simulink model "model_20ms"  (R2026a)
settings: Solver=VariableStepAuto
undefined symbols (not defined in the file): MIO, National_Instruments, PCI
libraries: sldrtlib x2, simulink x1
settings Model: Creator=acsdc  LastModifiedBy=acsdc

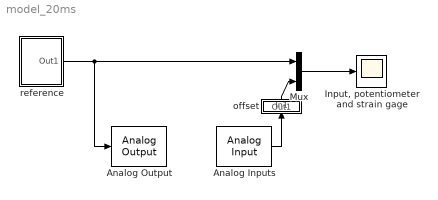
== system model_20ms ==
  Analog Inputs : sldrtlib/Analog Input  SampleTime=0.02  MaxMissedTicks=1000  ShowMissedTicks=off  YieldWhenWaiting=off  DrvName=National_Instruments/PCI-MIO-16E-4  DrvAddress=4294967295  DrvOptions=[0 0 0 0 0 0]  Channels=1:4  RangeMode=1  VoltRange=1  DataType=1
      settings: AttributesFormatString=National Instruments\nPCI-MIO-16E-4 [auto]
  Analog Output : sldrtlib/Analog Output  SampleTime=0.02  MaxMissedTicks=1000  ShowMissedTicks=off  YieldWhenWaiting=off  DrvName=National_Instruments/PCI-MIO-16E-4  DrvAddress=4294967295  DrvOptions=[0 0 0 0 0 0]  Channels=1  RangeMode=1  VoltRange=1  InitialValue=0  FinalValue=0
      settings: AttributesFormatString=National Instruments\nPCI-MIO-16E-4 [auto]
  "Input, potentiometer and strain gage" : Scope
      settings: DataLoggingSaveFormat=Array
  Mux : Mux  Inputs=2
  offset : Subsystem
  reference : Subsystem
  wires:
  Mux/1 -> "Input, potentiometer and strain gage"/1
  offset/1(Out1) -> Mux/2
  reference/1(Out1) -> Analog Output/1, Mux/1
  Analog Inputs/1 -> offset/1(In1)

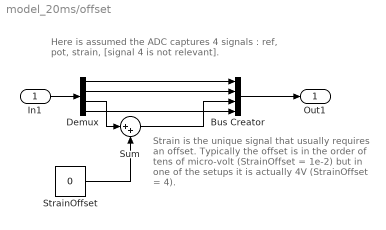
== system model_20ms/offset ==
  note: Strain is the unique signal that usually requires an offset. Typically the offset is in the order of tens of micro-volt (StrainOffset = 1e-2) but in one of the setups it is actually 4V (StrainOffset = 4).
  note: Here is assumed the ADC captures 4 signals :
      | ref, pot, strain, [signal 4 is not relevant].
  In1 : Inport
  Bus Creator : BusCreator  Inputs=4
  Demux : Demux
  StrainOffset : Constant  Value=0
  Sum : Sum  Inputs=|++
  Out1 : Outport
  wires:
  In1/1 -> Demux/1
  Bus Creator/1 -> Out1/1
  Demux/1 -> Bus Creator/1
  Demux/2 -> Bus Creator/2
  Demux/4 -> Bus Creator/4
  Demux/3 -> Sum/1
  Sum/1 -> Bus Creator/3
  StrainOffset/1 -> Sum/2

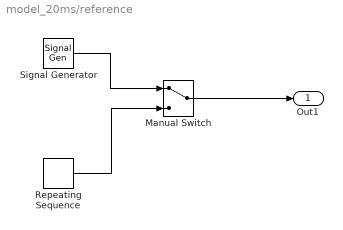
== system model_20ms/reference ==
  Manual Switch : ManualSwitch
  Repeating Sequence : simulink/Sources/Repeating Sequence  rep_seq_t=[0 0.9999 1 1.9999 2 2.9999 3 4]  rep_seq_y=[1 1 0 0 -1 -1 0 0]
  Signal Generator : SignalGenerator  WaveForm=square  Frequency=0.5
  Out1 : Outport
  wires:
  Signal Generator/1 -> Manual Switch/1
  Repeating Sequence/1 -> Manual Switch/2
  Manual Switch/1 -> Out1/1
